simulink model "drive_plant_foc"  (R2026b)
settings: Solver=VariableStepAuto
undefined symbols (not defined in the file or in its folder): P
libraries: nesl_utility x12, fl_lib x11, ee_lib x3, eeTransforms x2, eePmsmCurrentController x1, eePmsmCurrentReferenceGen x1, simulink x1
settings Model: Creator=aomar  LastModifiedBy=aomar

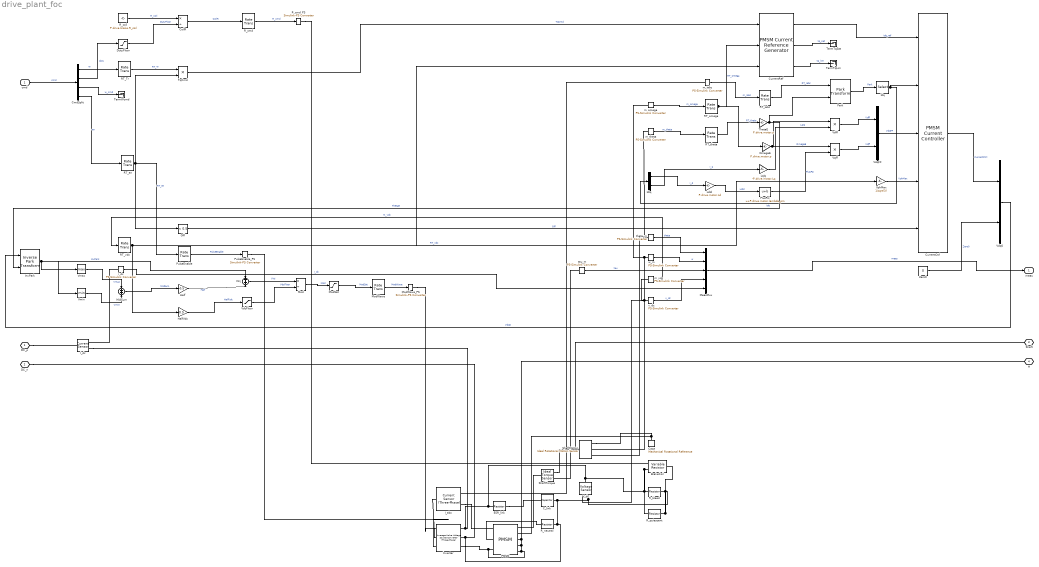
== system drive_plant_foc ==
  cmd : Inport  OutDataTypeStr=double  SampleTime=P.drive.Ts_esc
  BrakeCoil : fl_lib/Electrical/Electrical Elements/Variable Resistor  Rmin=1 Ohm  thermalEnable=false  thermal_mass=1 J/K  i_specify=off  i_priority=None  i=0 A  i_nominal_specify=off  i_nominal_value=1  i_nominal_unit=A  v_specify=off  v_priority=None  v=0 V  v_nominal_specify=off  v_nominal_value=1  v_nominal_unit=V  T_specify=off  T_priority=None  T=300 K  T_nominal_specify=off  T_nominal_value=1  T_nominal_unit=K
  C_link : fl_lib/Electrical/Electrical Elements/Capacitor  c=P.drive.esc.C_link F  r=1e-6 Ohm  g=0 1/Ohm  i_specify=off  i_priority=None  i=0 A  i_nominal_specify=off  i_nominal_value=1  i_nominal_unit=A  v_specify=off  v_priority=None  v=0 V  v_nominal_specify=off  v_nominal_value=1  v_nominal_unit=V  vc_specify=on  vc_priority=High  vc=P.drive.esc.vc0 V  vc_nominal_specify=off  vc_nominal_value=1  vc_nominal_unit=V
  Case : fl_lib/Mechanical/Rotational Elements/Mechanical Rotational Reference
  CmdSplit : Demux
  CoilR : Product  Inputs=*/
  CurrentCtrl : eePmsmCurrentController/PMSM Current Controller  Kp_id=P.drive.foc.Kp_i  Ki_id=P.drive.foc.Ki_i  Kaw_id=1  Kp_iq=P.drive.foc.Kp_i  Ki_iq=P.drive.foc.Ki_i  Kaw_iq=1  Ts=P.drive.Ts_foc  Tsd=P.drive.Ts_foc  AxisPrio=Q-axis  ActZC=off  ActFF=on
      settings: LibrarySourceBlock=ee_sl_lib/PMSM Control/PMSM Current Controller
  CurrentRef : eePmsmCurrentReferenceGen/PMSM Current Reference Generator  Vnom=P.drive.motor.V_nom  Pmax=P.drive.foc.P_max  Tmax=P.drive.motor.T_peak  Ts=P.drive.Ts_foc  RefType=Zero d-axis control  rpmVec=[0, 3000]  TqVec=[-100, 0, 100]  VdcVec=[300, 350]  PWMMode=SVM: space vector modulation  ModFactor=1  idMatrix=zeros(2,3,2)  iqMatrix=zeros(2,3,2)  p=P.drive.motor.p  psim=P.drive.motor.lambda_pm  Ld=P.drive.motor.Ld  Lq=P.drive.motor.Lq  Rs=P.drive.motor.Rs  RefExpEnable=0
      settings: LibrarySourceBlock=|
      | ee_sl_lib/PMSM Control/PMSM Current Reference
      | Generator
  DutyFloor : Saturate  UpperLimit=1  LowerLimit=P.drive.brake.duty_min
  ESR_link : fl_lib/Electrical/Electrical Elements/Resistor  R=P.drive.esc.ESR_link Ohm  i_specify=off  i_priority=None  i=0 A  i_nominal_specify=off  i_nominal_value=1  i_nominal_unit=A  v_specify=off  v_priority=None  v=0 V  v_nominal_specify=off  v_nominal_value=1  v_nominal_unit=V
  Half : Gain  Gain=-0.5
  HalfVdc : Gain  Gain=0.5
  I_abc : ee_lib/Sensors & Transducers/Current Sensor (Three-Phase)  port_option=ee.enum.threePhasePort.composite
  I_dc : fl_lib/Electrical/Electrical Sensors/Current Sensor
  IdIq : Demux  Outputs=2
  Idq : Selector  InputPortWidth=3  IndexOptions=Index vector (dialog)  Indices=[1 2]  OutputSizes=1
  InvPark : eeTransforms/Inverse Park Transform  AxisAlignment=D-axis  PowerInvariant=off
      settings: LibrarySourceBlock=|
      | ee_sl_lib/Mathematical
      | Transforms/Inverse
      | Park Transform
  Inverter : ee_lib/Semiconductors & Converters/Converters/Average-Value Voltage Source Converter (Three-Phase)  port_option=ee.enum.threePhasePort.composite  enable_block_pulses_input=true  krec=0.01 Ohm  frequency_option=ee.enum.converters.frequency.variable  input_option=ee.enum.converters.inputOption.ModWave  FRated=60 Hz  losses_parameterization=ee.enum.converters.losses.profile  Pfixed=1 W  ks=0.01  kc1=1.7 V  kc2=0.01 Ohm  Ploss_vect=P.drive.foc.Ploss_vect W  Irms_vect=P.drive.foc.Irms_vect A  Vdc_nom=P.drive.motor.V_nom V  thermal_mass=P.drive.foc.thermal_mass_inv J/K  temperature_specify=on  temperature_priority=High  temperature=P.drive.thermal.T_amb0 K  temperature_nominal_specify=off  temperature_nominal_value=1  temperature_nominal_unit=K
  LdId : Gain  Gain=P.drive.motor.Ld
  LqIq : Gain  Gain=-P.drive.motor.Lq
  MeasMux : Mux  Inputs=5
  MidSum : Sum
  Mod : Product  Inputs=*/
  ModSat : Saturate  UpperLimit=1  LowerLimit=-1
  ModWave : RateTransition  OutPortSampleTimeOpt=Inherit
  ModWave_PS : nesl_utility/Simulink-PS Converter  PhysicalDomain=network_engine_domain  SubClassName=ps_input  LeftPortType=input  RightPortType=output  PseudoPeriodic=off  Frequencies=[]  NoiseDistribution=none  NoiseParameters=[]  Unit=1  AffineConversion=off  FilteringAndDerivatives=zero  SimscapeFilterOrder=1  InputFilterTimeConstant=0.001  UdotUserProvided=0
  Off : simulink/Logic and Bit Operations/Compare To Constant  relop=<  const=0.5  OutDataTypeStr=boolean
  OmegaE : Gain  Gain=P.drive.motor.p
  PMSM : ee_lib/Electromechanical/Permanent Magnet/PMSM  port_option=ee.enum.threePhasePort.composite  winding_type=ee.enum.electromech.statorconfiguration.wye  machine_param=ee.enum.pmsm.parameterization.constant  nPolePairs=P.drive.motor.p  pmflux_param=ee.enum.pmflux.fluxlinkage  pm_flux_linkage=P.drive.motor.lambda_pm Wb  torque_constant=0.18 N*m/A  back_emf_constant=0.18 V*s/rad  stator_param=ee.enum.statorparam.LdLqL0  Ld=P.drive.motor.Ld H  Lq=P.drive.motor.Lq H  idVec=[-200, 0, 200] A  iqVec=[-200, 0, 200] A  LdMatrix=0.0002 * ones(3, 3) H  LqMatrix=0.0002 * ones(3, 3) H  PmMatrix=0.1 * ones(3, 3) Wb  ktMatrix=0.18 * ones(3, 3) N*m/A  keMatrix=0.18 * ones(3, 3) V*s/rad  L0=P.drive.motor.L0 H  Ls=0.0002 H  Lm=-0.00002 H  Ms=0.00002 H  Rs=P.drive.motor.Rs Ohm  zero_sequence=ee.enum.park.zerosequence.include  axes_param=ee.enum.rotorangle.daxis  loss_param=ee.enum.ironloss.empirical  losses_oc=P.drive.foc.losses_oc W  losses_sc=[0 0 0] W  f_losses=P.drive.foc.f_losses Hz  Isc_losses=95 A  J=P.drive.motor.J kg*m^2  lam=P.drive.motor.lam N*m*s/rad  i_d_specify=off  i_d_priority=None  i_d=0 A  i_d_nominal_specify=off  i_d_nominal_value=1  i_d_nominal_unit=A  i_q_specify=off  i_q_priority=None  i_q=0 A  i_q_nominal_specify=off  i_q_nominal_value=1  i_q_nominal_unit=A  torque_specify=off  torque_priority=None  torque=0 N*m  torque_nominal_specify=off  torque_nominal_value=1  torque_nominal_unit=N*m  angular_velocity_specify=off  angular_velocity_priority=High  angular_velocity=0 rpm  angular_velocity_nominal_specify=off  angular_velocity_nominal_value=1  angular_velocity_nominal_unit=rpm  angular_position_specify=off  angular_position_priority=High  angular_position=0 deg  angular_position_nominal_specify=off  angular_position_nominal_value=1  angular_position_nominal_unit=deg  alpha=P.drive.motor.alpha_cu 1/K  alpha_flux=-0.001 1/K  Tmeas=298.15 K  stator_thermal_mass=P.drive.foc.C_stator J/K  rotor_thermal_mass=P.drive.foc.C_rotor J/K  Rm_percent_rotor=90  Rd_percent_rotor=30  temperatureA_specify=on  temperatureA_priority=High  temperatureA=P.drive.thermal.T_amb0 K  temperatureA_nominal_specify=off  temperatureA_nominal_value=1  temperatureA_nominal_unit=degC  temperatureB_specify=on  temperatureB_priority=High  temperatureB=P.drive.thermal.T_amb0 K  temperatureB_nominal_specify=off  temperatureB_nominal_value=1  temperatureB_nominal_unit=degC  temperatureC_specify=on  temperatureC_priority=High  temperatureC=P.drive.thermal.T_amb0 K  temperatureC_nominal_specify=off  temperatureC_nominal_value=1  temperatureC_nominal_unit=degC  temperatureR_specify=on  temperatureR_priority=High  temperatureR=P.drive.thermal.T_amb0 K  temperatureR_nominal_specify=off  temperatureR_nominal_value=1  temperatureR_nominal_unit=degC
  Park : eeTransforms/Park Transform  AxisAlignment=D-axis  PowerInvariant=off
      settings: LibrarySourceBlock=|
      | ee_sl_lib/Mathematical
      | Transforms/Park Transform
  PlusPsi : Bias  Bias=P.drive.motor.lambda_pm  SaturateOnIntegerOverflow=off
  PulseEnable : RateTransition  OutPortSampleTimeOpt=Inherit
  PulseEnable_PS : nesl_utility/Simulink-PS Converter  PhysicalDomain=network_engine_domain  SubClassName=ps_input  LeftPortType=input  RightPortType=output  PseudoPeriodic=off  Frequencies=[]  NoiseDistribution=none  NoiseParameters=[]  Unit=1  AffineConversion=off  FilteringAndDerivatives=zero  SimscapeFilterOrder=1  InputFilterTimeConstant=0.001  UdotUserProvided=0
  RT_Tr : RateTransition  OutPortSampleTime=P.drive.Ts_foc
  RT_en : RateTransition  OutPortSampleTime=P.drive.Ts_foc
  RT_iabc : RateTransition  OutPortSampleTime=P.drive.Ts_foc
  RT_omega : RateTransition  OutPortSampleTime=P.drive.Ts_foc
  RT_theta : RateTransition  OutPortSampleTime=P.drive.Ts_foc
  RT_vdc : RateTransition  OutPortSampleTime=P.drive.Ts_foc
  R_bleed : fl_lib/Electrical/Electrical Elements/Resistor  R=P.drive.esc.R_bleed Ohm  i_specify=off  i_priority=None  i=0 A  i_nominal_specify=off  i_nominal_value=1  i_nominal_unit=A  v_specify=off  v_priority=None  v=0 V  v_nominal_specify=off  v_nominal_value=1  v_nominal_unit=V
  R_cmd : RateTransition  OutPortSampleTimeOpt=Inherit
  R_cmd_PS : nesl_utility/Simulink-PS Converter  PhysicalDomain=network_engine_domain  SubClassName=ps_input  LeftPortType=input  RightPortType=output  PseudoPeriodic=off  Frequencies=[]  NoiseDistribution=none  NoiseParameters=[]  Unit=Ohm  AffineConversion=off  FilteringAndDerivatives=zero  SimscapeFilterOrder=1  InputFilterTimeConstant=0.001  UdotUserProvided=0
  R_coil : Constant  Value=P.drive.brake.R_coil
  R_neutral : fl_lib/Electrical/Electrical Elements/Resistor  R=P.drive.tie.R Ohm  i_specify=off  i_priority=None  i=0 A  i_nominal_specify=off  i_nominal_value=1  i_nominal_unit=A  v_specify=off  v_priority=None  v=0 V  v_nominal_specify=off  v_nominal_value=1  v_nominal_unit=V
  R_quiescent : fl_lib/Electrical/Electrical Elements/Resistor  R=P.drive.esc.R_q Ohm  i_specify=off  i_priority=None  i=0 A  i_nominal_specify=off  i_nominal_value=1  i_nominal_unit=A  v_specify=off  v_priority=None  v=0 V  v_nominal_specify=off  v_nominal_value=1  v_nominal_unit=V
  ShaftMotion : fl_lib/Mechanical/Mechanical Sensors/Ideal Rotational Motion Sensor  reference=foundation.enum.MeasurementReference.difference  acceleration_port=false  velocity_port=true  position_port=true  wrap_angle=false  offset=0 rad
  ShaftTorque : fl_lib/Mechanical/Mechanical Sensors/Ideal Torque Sensor
  TermTqLim : Terminator
  TermTqSat : Terminator
  TermWcmd : Terminator
  ThetaE : Gain  Gain=P.drive.motor.p
  TqCmd : Product  Inputs=**
  VInj : Sum
  V_dc : fl_lib/Electrical/Electrical Sensors/Voltage Sensor
  VdcFloor : Saturate  UpperLimit=inf  LowerLimit=1
  Vdff : Product  Inputs=**
  Vdq0 : Mux  Inputs=2
  VdqFF : Mux  Inputs=2
  Vmax : MinMax  Function=max
  Vmin : MinMax
  VphMax : Gain  Gain=1/sqrt(3)
  Vqff : Product  Inputs=**
  Zero0 : Constant  Value=0
  i_dc : nesl_utility/PS-Simulink Converter  PhysicalDomain=network_engine_domain  SubClassName=ps_output  LeftPortType=input  RightPortType=output  PseudoPeriodic=off  Frequencies=[]  VectorFormat=inherit  Unit=A  AffineConversion=off
  m_iabc : nesl_utility/PS-Simulink Converter  PhysicalDomain=network_engine_domain  SubClassName=ps_output  LeftPortType=input  RightPortType=output  PseudoPeriodic=off  Frequencies=[]  VectorFormat=inherit  Unit=A  AffineConversion=off
  m_omega : nesl_utility/PS-Simulink Converter  PhysicalDomain=network_engine_domain  SubClassName=ps_output  LeftPortType=input  RightPortType=output  PseudoPeriodic=off  Frequencies=[]  VectorFormat=inherit  Unit=rad/s  AffineConversion=off
  m_theta : nesl_utility/PS-Simulink Converter  PhysicalDomain=network_engine_domain  SubClassName=ps_output  LeftPortType=input  RightPortType=output  PseudoPeriodic=off  Frequencies=[]  VectorFormat=inherit  Unit=rad  AffineConversion=off
  m_vdc : nesl_utility/PS-Simulink Converter  PhysicalDomain=network_engine_domain  SubClassName=ps_output  LeftPortType=input  RightPortType=output  PseudoPeriodic=off  Frequencies=[]  VectorFormat=inherit  Unit=V  AffineConversion=off
  tau_m : nesl_utility/PS-Simulink Converter  PhysicalDomain=network_engine_domain  SubClassName=ps_output  LeftPortType=input  RightPortType=output  PseudoPeriodic=off  Frequencies=[]  VectorFormat=inherit  Unit=N*m  AffineConversion=off
  theta_m : nesl_utility/PS-Simulink Converter  PhysicalDomain=network_engine_domain  SubClassName=ps_output  LeftPortType=input  RightPortType=output  PseudoPeriodic=off  Frequencies=[]  VectorFormat=inherit  Unit=rad  AffineConversion=off
  v_dc : nesl_utility/PS-Simulink Converter  PhysicalDomain=network_engine_domain  SubClassName=ps_output  LeftPortType=input  RightPortType=output  PseudoPeriodic=off  Frequencies=[]  VectorFormat=inherit  Unit=V  AffineConversion=off
  w_m : nesl_utility/PS-Simulink Converter  PhysicalDomain=network_engine_domain  SubClassName=ps_output  LeftPortType=input  RightPortType=output  PseudoPeriodic=off  Frequencies=[]  VectorFormat=inherit  Unit=rad/s  AffineConversion=off
  DC_p : PMIOPort  Side=Left  ConnectionType=Connection: foundation.electrical.electrical
  DC_n : PMIOPort  Port=2  Side=Left  ConnectionType=Connection: foundation.electrical.electrical
  Shaft : PMIOPort  Port=3  Side=Right  ConnectionType=Connection: foundation.mechanical.rotational.rotational
  H : PMIOPort  Port=4  Side=Right  ConnectionType=Connection: foundation.thermal.thermal
  meas : Outport  OutDataTypeStr=double
  wires:
  cmd/1 -> CmdSplit/1  "cmd"
  InvPark/1 -> Vmin/1, VInj/1, Vmax/1  "InvPark"
  CmdSplit/1 -> RT_Tr/1  "Tr"
  CmdSplit/2 -> DutyFloor/1  "duty"
  CmdSplit/3 -> TermWcmd/1  "w_cmd"
  CmdSplit/4 -> RT_en/1  "en"
  Vmax/1 -> MidSum/1  "Vmax"
  Vmin/1 -> MidSum/2  "Vmin"
  i_dc/1 -> MeasMux/5  "i_dc"
  MidSum/1 -> Half/1  "MidSum"
  R_coil/1 -> CoilR/1  "R_coil"
  DutyFloor/1 -> CoilR/2  "DutyFloor"
  RT_Tr/1 -> TqCmd/1  "RT_Tr"
  RT_vdc/1 -> CurrentRef/3, HalfVdc/1, VphMax/1  "RT_vdc"
  RT_en/1 -> PulseEnable/1, TqCmd/2, Off/1  "RT_en"
  CoilR/1 -> R_cmd/1  "CoilR"
  TqCmd/1 -> CurrentRef/1  "TqCmd"
  Off/1 -> CurrentCtrl/5  "Off"
  Half/1 -> VInj/2  "Half"
  HalfVdc/1 -> VdcFloor/1  "HalfVdc"
  PulseEnable/1 -> PulseEnable_PS/1  "PulseEnable"
  VInj/1 -> Mod/1  "VInj"
  VdcFloor/1 -> Mod/2  "VdcFloor"
  R_cmd/1 -> R_cmd_PS/1  "R_cmd"
  Mod/1 -> ModSat/1  "Mod"
  ModSat/1 -> ModWave/1  "ModSat"
  ModWave/1 -> ModWave_PS/1  "ModWave"
  tau_m/1 -> MeasMux/3  "tau"
  IdIq/1 -> LdId/1  "i_d"
  IdIq/2 -> LqIq/1  "i_q"
  m_omega/1 -> RT_omega/1  "m_omega"
  m_theta/1 -> RT_theta/1  "m_theta"
  theta_m/1 -> MeasMux/1  "theta"
  w_m/1 -> MeasMux/2  "w"
  m_vdc/1 -> RT_vdc/1  "m_vdc"
  v_dc/1 -> MeasMux/4  "v_dc"
  MeasMux/1 -> meas/1  "meas"
  m_iabc/1 -> RT_iabc/1  "m_iabc"
  LdId/1 -> PlusPsi/1  "LdId"
  RT_omega/1 -> CurrentRef/2, OmegaE/1  "RT_omega"
  RT_theta/1 -> ThetaE/1  "RT_theta"
  ThetaE/1 -> InvPark/2, Park/2  "ThetaE"
  LqIq/1 -> Vdff/2  "LqIq"
  RT_iabc/1 -> Park/1  "RT_iabc"
  OmegaE/1 -> Vdff/1, Vqff/1  "OmegaE"
  PlusPsi/1 -> Vqff/2  "PlusPsi"
  CurrentRef/1 -> CurrentCtrl/1  "idq_ref"
  CurrentRef/2 -> TermTqSat/1  "tq_sat"
  CurrentRef/3 -> TermTqLim/1  "tq_lim"
  Vdff/1 -> VdqFF/1  "Vdff"
  Vqff/1 -> VdqFF/2  "Vqff"
  Park/1 -> Idq/1  "Park"
  VdqFF/1 -> CurrentCtrl/3  "VdqFF"
  VphMax/1 -> CurrentCtrl/4  "VphMax"
  Idq/1 -> IdIq/1, CurrentCtrl/2  "Idq"
  Zero0/1 -> Vdq0/2  "Zero0"
  CurrentCtrl/1 -> Vdq0/1  "CurrentCtrl"
  Vdq0/1 -> InvPark/1  "Vdq0"
  connections:
  R_cmd_PS/RConn1 -- BrakeCoil/LConn1
  Inverter/RConn1 -- I_dc/RConn2 -- ESR_link/LConn1 -- V_dc/LConn1 -- R_bleed/LConn1 -- BrakeCoil/LConn2 -- R_quiescent/LConn1
  Inverter/RConn2 -- DC_n/RConn1 -- R_neutral/RConn1 -- C_link/RConn1 -- V_dc/RConn2 -- R_bleed/RConn1 -- R_quiescent/RConn1 -- BrakeCoil/RConn1
  ESR_link/RConn1 -- C_link/LConn1
  Case/LConn1 -- ShaftMotion/RConn1 -- PMSM/RConn2
  DC_p/RConn1 -- I_dc/LConn1
  PMSM/LConn3 -- Inverter/RConn3 -- PMSM/RConn5 -- PMSM/RConn4 -- PMSM/RConn3 -- H/RConn1
  I_abc/LConn1 -- Inverter/LConn2
  m_iabc/LConn1 -- I_abc/RConn1
  I_abc/RConn2 -- PMSM/LConn1
  i_dc/LConn1 -- I_dc/RConn1
  ModWave_PS/RConn1 -- Inverter/LConn1
  PulseEnable_PS/RConn1 -- Inverter/LConn3
  PMSM/LConn2 -- R_neutral/LConn1
  ShaftTorque/LConn1 -- PMSM/RConn1
  ShaftMotion/LConn1 -- ShaftTorque/RConn1 -- Shaft/RConn1
  w_m/LConn1 -- m_omega/LConn1 -- ShaftMotion/RConn2
  theta_m/LConn1 -- m_theta/LConn1 -- ShaftMotion/RConn3
  tau_m/LConn1 -- ShaftTorque/RConn2
  v_dc/LConn1 -- m_vdc/LConn1 -- V_dc/RConn1
